simulink model "trimNonlinearAirframe"  (R2026a)
settings: Solver=ode3  StartTime=0  StopTime=100  FixedStep=Ts  EnableMultiTasking=on
settings Model: Creator=The MathWorks, Inc.  LastModifiedBy=The MathWorks, Inc.
settings DataIOCC: ExternalInput=getinputstruct(op)  InitialState=getstatestruct(op)  SaveFormat=StructureWithTime
settings OptimizationCC: BufferReuse=off
settings DebuggingCC: UnderspecifiedInitializationDetection=Classic
settings HardwareCC: ProdHWDeviceType=32-bit Generic

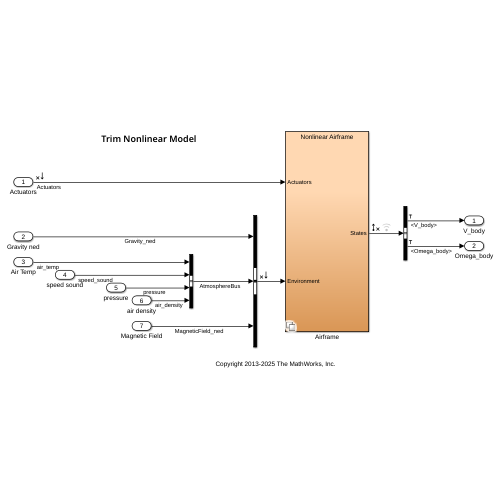
[thumbnail: Simulink's stored preview of the top-level diagram]
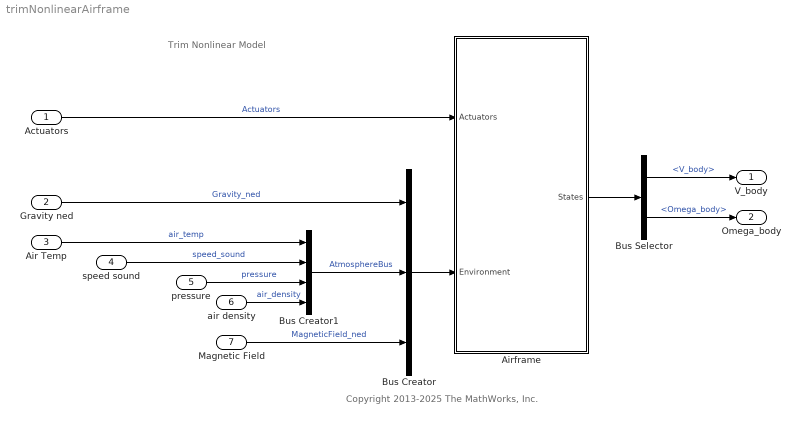
== system trimNonlinearAirframe ==
  note: Trim Nonlinear Model
  note: Copyright 2013-2025 The MathWorks, Inc.
  Actuators : Inport  PortDimensions=[1 4]
  Gravity ned : Inport  Port=2
  Air Temp : Inport  Port=3
  speed sound : Inport  Port=4
  pressure : Inport  Port=5
  air density : Inport  Port=6
  Magnetic Field : Inport  Port=7
  Airframe : Subsystem  Variant=on
  Bus Creator : BusCreator  Inputs=3  OutDataTypeStr=Bus: EnvironmentBus  NonVirtualBus=on
  Bus Creator1 : BusCreator  Inputs=4  OutDataTypeStr=Bus: AtmosphereBus  NonVirtualBus=on
  Bus Selector : BusSelector  OutputSignals=V_body,Omega_body
  V_body : Outport  VectorParamsAs1DForOutWhenUnconnected=off
  Omega_body : Outport  Port=2  VectorParamsAs1DForOutWhenUnconnected=off
  wires:
  Actuators/1 -> Airframe/1(Actuators)  "Actuators"
  Airframe/1(States) -> Bus Selector/1
  Magnetic Field/1 -> Bus Creator/3  "MagneticField_ned"
  Bus Creator1/1 -> Bus Creator/2  "AtmosphereBus"
  air density/1 -> Bus Creator1/4  "air_density"
  pressure/1 -> Bus Creator1/3  "pressure"
  speed sound/1 -> Bus Creator1/2  "speed_sound"
  Air Temp/1 -> Bus Creator1/1  "air_temp"
  Bus Creator/1 -> Airframe/2(Environment)
  Gravity ned/1 -> Bus Creator/1  "Gravity_ned"
  Bus Selector/1 -> V_body/1  "<V_body>"
  Bus Selector/2 -> Omega_body/1  "<Omega_body>"

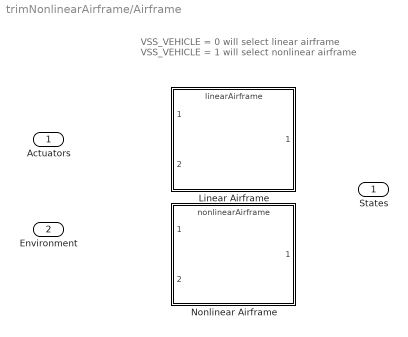
== system trimNonlinearAirframe/Airframe ==
  note: VSS_VEHICLE = 0 will select linear airframe
      | VSS_VEHICLE = 1 will select nonlinear airframe
  Actuators : Inport
  Environment : Inport  Port=2  OutDataTypeStr=Bus: EnvironmentBus
  Linear Airframe : ModelReference  ModelNameDialog=linearAirframe.slx  SimulationMode=Normal  VariantControl=VSS_VEHICLE_LINEAR  ModelReferenceVersion=5.0
  Nonlinear Airframe : ModelReference  ModelNameDialog=nonlinearAirframe.slx  SimulationMode=Normal  VariantControl=VSS_VEHICLE_NONLINEAR  ModelReferenceVersion=13.0
  States : Outport  OutDataTypeStr=Bus: StatesBus  VectorParamsAs1DForOutWhenUnconnected=off
